simulink model "headroom"  (R2026a)
settings: Solver=VariableStepAuto  StopTime=0.0001
libraries: hdlsllib x10, dsphdlsigops2 x1
settings Model: Creator=taokhe  LastModifiedBy=taokhe

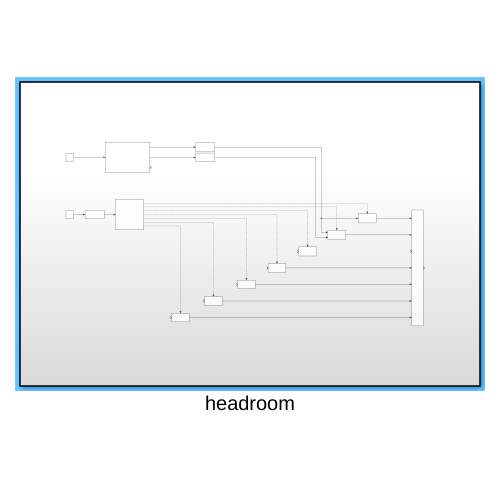
[thumbnail: Simulink's stored preview of the top-level diagram]
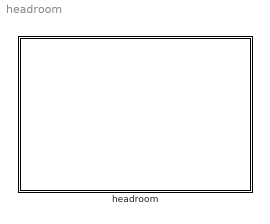
== system headroom ==
  headroom : Subsystem

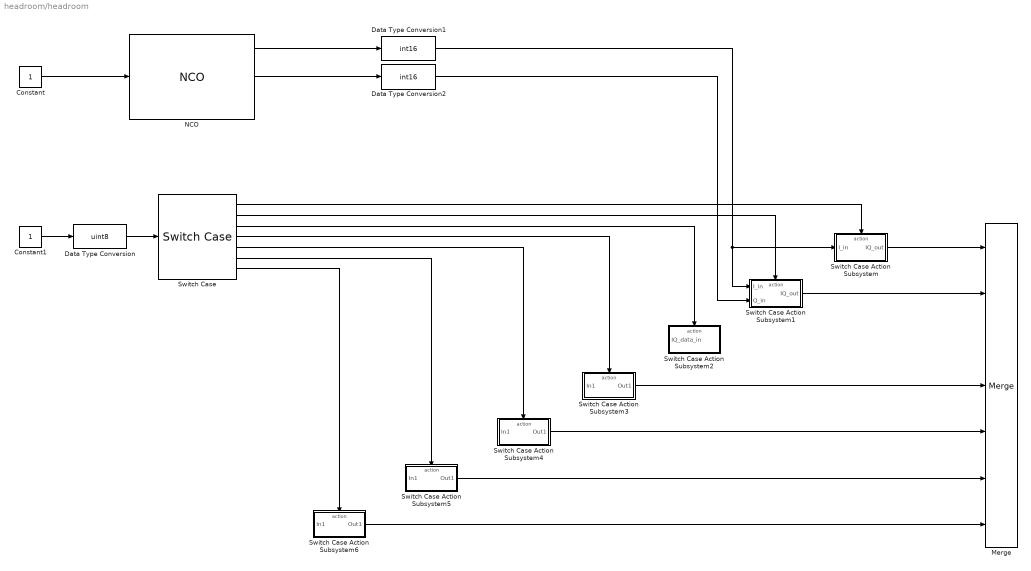
== system headroom/headroom ==
  Constant : Constant  OutDataTypeStr=boolean  SampleTime=1/250e6
  Constant1 : Constant
  Data Type Conversion : DataTypeConversion  OutDataTypeStr=uint8  SaturateOnIntegerOverflow=off  RndMeth=Floor
  Data Type Conversion1 : DataTypeConversion  OutDataTypeStr=int16  ConvertRealWorld=Stored Integer (SI)  SaturateOnIntegerOverflow=off  RndMeth=Floor
  Data Type Conversion2 : DataTypeConversion  OutDataTypeStr=int16  ConvertRealWorld=Stored Integer (SI)  SaturateOnIntegerOverflow=off  RndMeth=Floor
  Merge : Merge  Inputs=7
  NCO : dsphdlsigops2/NCO  PhaseIncrementSource=Property  PhaseIncrement=85899346  Frequency=510  FreqResolution=0.05  SamplingFreq=4000  PhaseOffsetSource=Property  PhaseOffset=1.0737e+09  PhaseOffsetR=pi/3  DitherSource=Property  NumDitherBits=13  SamplesPerFrame=1  LUTCompress=off  ResetAction=off  Waveform=Sine and cosine  PhasePort=off  SimulateUsing=Code generation  AccumulatorWL=32  PhaseQuantization=on  NumQuantizerAccumulatorBits=19  OutputDataType=Binary point scaling  OutputWL=16  OutputFL=15
  Switch Case : SwitchCase  CaseConditions={0, 1, 2, 3, 4, 5}
  Switch Case Action Subsystem : Subsystem  TreatAsAtomicUnit=on
  Switch Case Action Subsystem1 : Subsystem  TreatAsAtomicUnit=on
  Switch Case Action Subsystem2 : Subsystem  TreatAsAtomicUnit=on
  Switch Case Action Subsystem3 : Subsystem  TreatAsAtomicUnit=on
  Switch Case Action Subsystem4 : Subsystem  TreatAsAtomicUnit=on
  Switch Case Action Subsystem5 : Subsystem  TreatAsAtomicUnit=on
  Switch Case Action Subsystem6 : Subsystem  TreatAsAtomicUnit=on
  wires:
  Constant1/1 -> Data Type Conversion/1
  Data Type Conversion/1 -> Switch Case/1
  Switch Case/1 -> Switch Case Action Subsystem/Action
  Switch Case/2 -> Switch Case Action Subsystem1/Action
  Switch Case/3 -> Switch Case Action Subsystem2/Action
  Switch Case/4 -> Switch Case Action Subsystem3/Action
  Switch Case/5 -> Switch Case Action Subsystem4/Action
  Switch Case/6 -> Switch Case Action Subsystem5/Action
  Switch Case/7 -> Switch Case Action Subsystem6/Action
  Switch Case Action Subsystem3/1(Out1) -> Merge/4
  Switch Case Action Subsystem4/1(Out1) -> Merge/5
  Switch Case Action Subsystem5/1(Out1) -> Merge/6
  Switch Case Action Subsystem6/1(Out1) -> Merge/7
  Constant/1 -> NCO/1
  NCO/1 -> Data Type Conversion1/1
  NCO/2 -> Data Type Conversion2/1
  Switch Case Action Subsystem/1(IQ_out) -> Merge/1
  Switch Case Action Subsystem1/1(IQ_out) -> Merge/2
  Data Type Conversion1/1 -> Switch Case Action Subsystem1/1("I_in "), Switch Case Action Subsystem/1("I_in ")
  Data Type Conversion2/1 -> Switch Case Action Subsystem1/2("Q_in ")

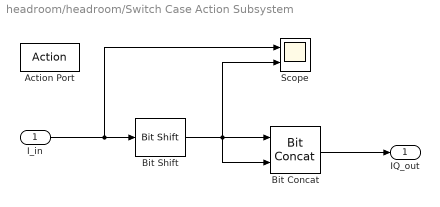
== system headroom/headroom/Switch Case Action Subsystem ==
  "I_in " : Inport
  Action Port : ActionPort  ActionPortLabel=case [ 0 ]:
  Bit Concat : hdlsllib/Logic and Bit Operations/Bit Concat  numInputs=2
  Bit Shift : hdlsllib/Logic and Bit Operations/Bit Shift  mode=Shift Right Arithmetic  N=2
  Scope : Scope  NumInputPorts=2
  IQ_out : Outport
  wires:
  Bit Shift/1 -> Scope/2, Bit Concat/2, Bit Concat/1
  "I_in "/1 -> Scope/1, Bit Shift/1
  Bit Concat/1 -> IQ_out/1

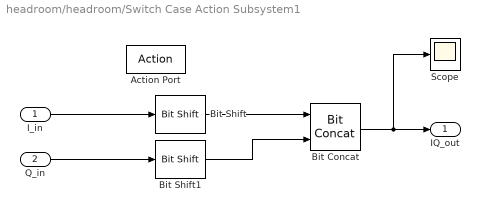
== system headroom/headroom/Switch Case Action Subsystem1 ==
  "I_in " : Inport
  "Q_in " : Inport  Port=2
  Action Port : ActionPort  ActionPortLabel=case [ 1 ]:
  Bit Concat : hdlsllib/Logic and Bit Operations/Bit Concat  numInputs=2
  Bit Shift : hdlsllib/Logic and Bit Operations/Bit Shift  mode=Shift Right Arithmetic  N=2
  Bit Shift1 : hdlsllib/Logic and Bit Operations/Bit Shift  mode=Shift Right Arithmetic  N=2
  Scope : Scope
      settings: ActiveDisplayYMinimum=-5.3266739399999988E+8  ActiveDisplayYMaximum=4.794006546E+9
  IQ_out : Outport
  wires:
  "I_in "/1 -> Bit Shift/1
  "Q_in "/1 -> Bit Shift1/1
  Bit Concat/1 -> Scope/1, IQ_out/1
  Bit Shift/1 -> Bit Concat/1
  Bit Shift1/1 -> Bit Concat/2

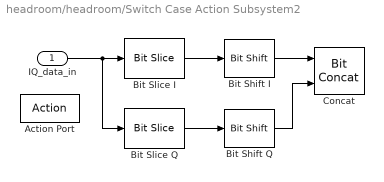
== system headroom/headroom/Switch Case Action Subsystem2 ==
  IQ_data_in : Inport  OutDataTypeStr=uint32
  Action Port : ActionPort  ActionPortLabel=case [ 2 ]:
  Bit Shift I : hdlsllib/Logic and Bit Operations/Bit Shift  mode=Shift Right Arithmetic  N=2
  Bit Shift Q : hdlsllib/Logic and Bit Operations/Bit Shift  mode=Shift Right Arithmetic  N=2
  Bit Slice I : hdlsllib/Logic and Bit Operations/Bit Slice  lidx=31  ridx=16
  Bit Slice Q : hdlsllib/Logic and Bit Operations/Bit Slice  lidx=15  ridx=0
  Concat : hdlsllib/Logic and Bit Operations/Bit Concat  numInputs=2
  wires:
  Bit Shift Q/1 -> Concat/2
  Bit Shift I/1 -> Concat/1
  Bit Slice Q/1 -> Bit Shift Q/1
  Bit Slice I/1 -> Bit Shift I/1
  IQ_data_in/1 -> Bit Slice I/1, Bit Slice Q/1

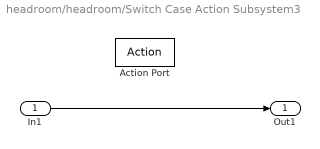
== system headroom/headroom/Switch Case Action Subsystem3 ==
  In1 : Inport
  Action Port : ActionPort  ActionPortLabel=case [ 3 ]:
  Out1 : Outport
  wires:
  In1/1 -> Out1/1

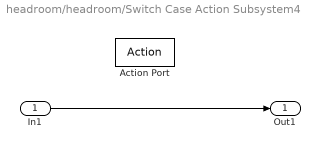
== system headroom/headroom/Switch Case Action Subsystem4 ==
  In1 : Inport
  Action Port : ActionPort  ActionPortLabel=case [ 4 ]:
  Out1 : Outport
  wires:
  In1/1 -> Out1/1

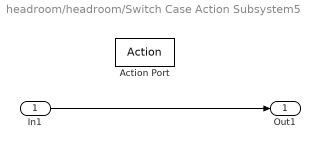
== system headroom/headroom/Switch Case Action Subsystem5 ==
  In1 : Inport
  Action Port : ActionPort  ActionPortLabel=case [ 5 ]:
  Out1 : Outport
  wires:
  In1/1 -> Out1/1

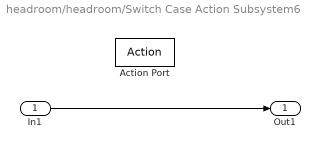
== system headroom/headroom/Switch Case Action Subsystem6 ==
  In1 : Inport
  Action Port : ActionPort  ActionPortLabel=default:
  Out1 : Outport
  wires:
  In1/1 -> Out1/1
